simulink model "test_phase_shift_filter"  (R2025b)
settings: Solver=ode1  StartTime=0.0  StopTime=1  FixedStep=ts_inv  RelTol=1e-3
values from neighbouring files (symbols this model uses):
  frequency_set = 300    [init_model_legacy.m]
undefined symbols (not defined in the file or in its folder): ts_inv
libraries: phase_shift_filter x1
settings Model: SimulationMode=accelerator  Creator=dbagn  LastModifiedBy=dbagn
settings SFSimCC: SimCustomHeaderCode=|
  | #include "rpi.h"
  | #include "mavgflt.h"
  | #include "mavgflt_simulink.h"
  | #include "mavgflts.h"
  | #include "mavgflts_simulink.h"
  | #include "dsmavgflt.h"
  | #include "dsmavgflt_simulink.h"
  | #include "bemf_obsv.h"
  | #include "bemf_obsv_simulink.h"
  | #include "bemf_obsv_load_est.h"
  | #include "bemf_obsv_load_est_simulink.h"
  | #include "dqvector_pi.h"
  | #include "dqvector_pi_simulink.h"
  | #include "sv_pwm_simulink.h"
  | #include "sv_pwm.h"
  | #include "first_harmonic_tracker.h"
  | #include "first_harmonic_tracker_simulink.h"
  | #include "dqpll_thyr.h"
  | #include "dqpll_thyr_simulink.h"
  | #include "dqpll_grid.h"
  | #include "dqpll_grid_simulink.h"
  | #include "phase_shift_flt_simulink.h"
  | #include "phase_shift_flt.h"
settings SFSimCC: SimUserSources=|
  | "rpi.c"
  | "mavgflt_simulink.c"
  | "mavgflt.c"
  | "mavgflts_simulink.c"
  | "mavgflts.c"
  | "dsmavgflt_simulink.c"
  | "dsmavgflt.c"
  | "bemf_obsv_simulink.c"
  | "bemf_obsv.c"
  | "bemf_obsv_load_est_simulink.c"
  | "bemf_obsv_load_est.c"
  | "dqvector_pi.c"
  | "dqvector_pi_simulink.c"
  | "sv_pwm_simulink.c"
  | "sv_pwm.c"
  | "first_harmonic_tracker_simulink.c"
  | "first_harmonic_tracker.c"
  | "dqpll_thyr_simulink.c"
  | "dqpll_thyr.c"
  | "dqpll_grid_simulink.c"
  | "dqpll_grid.c"
  | "phase_shift_flt_simulink.c"
  | "phase_shift_flt.c"
settings SFSimCC: SimUserIncludeDirs=|
  | include
  | src

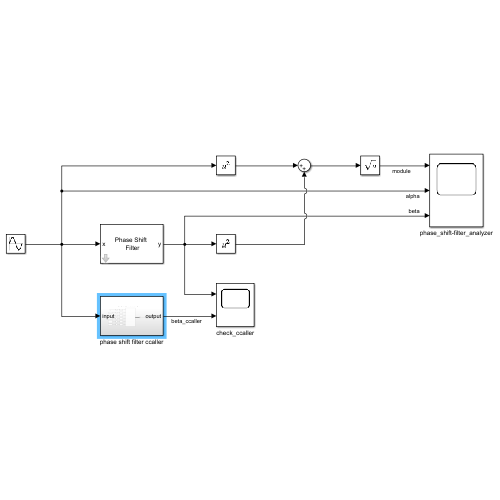
[thumbnail: Simulink's stored preview of the top-level diagram]
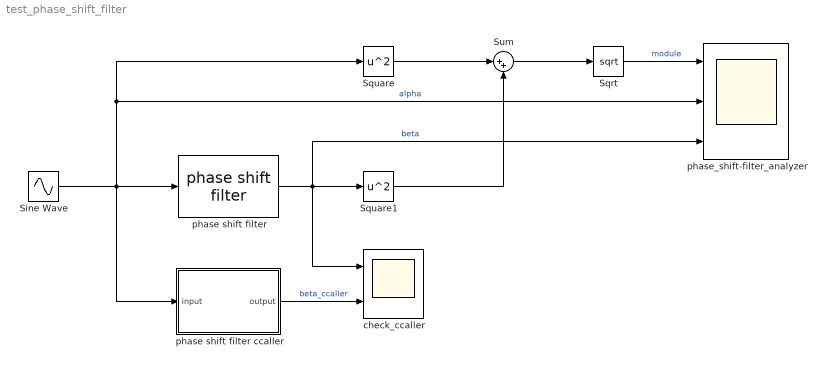
== system test_phase_shift_filter ==
  Sine Wave : Sin  Frequency=frequency_set*2*pi  SampleTime=0
  Sqrt : Sqrt
  Square : Math  Operator=square
  Square1 : Math  Operator=square
  Sum : Sum  Inputs=|++
  check_ccaller : Scope  NumInputPorts=2
      settings: SampleTime=ts_inv  ActiveDisplayYMinimum=-1.2559883330074681  ActiveDisplayYMaximum=1.2979435207382621
  phase shift filter : phase_shift_filter/phase shift filter  f=frequency_set  scaling_factor=phase_shift_filter_gain  ts=ts_inv
  phase shift filter ccaller : Subsystem
  phase_shift-filter_analyzer : Scope  NumInputPorts=3
      settings: SampleTime=ts_inv  ActiveDisplayYMinimum=-1.1297586136004538  ActiveDisplayYMaximum=1.507573484556453
  wires:
  Sine Wave/1 -> phase shift filter ccaller/1(input), Square/1, phase_shift-filter_analyzer/2, phase shift filter/1  "alpha"
  phase shift filter/1 -> check_ccaller/1, phase_shift-filter_analyzer/3, Square1/1  "beta"
  Square/1 -> Sum/1
  Square1/1 -> Sum/2
  Sum/1 -> Sqrt/1
  Sqrt/1 -> phase_shift-filter_analyzer/1  "module"
  phase shift filter ccaller/1(output) -> check_ccaller/2  "beta_ccaller"

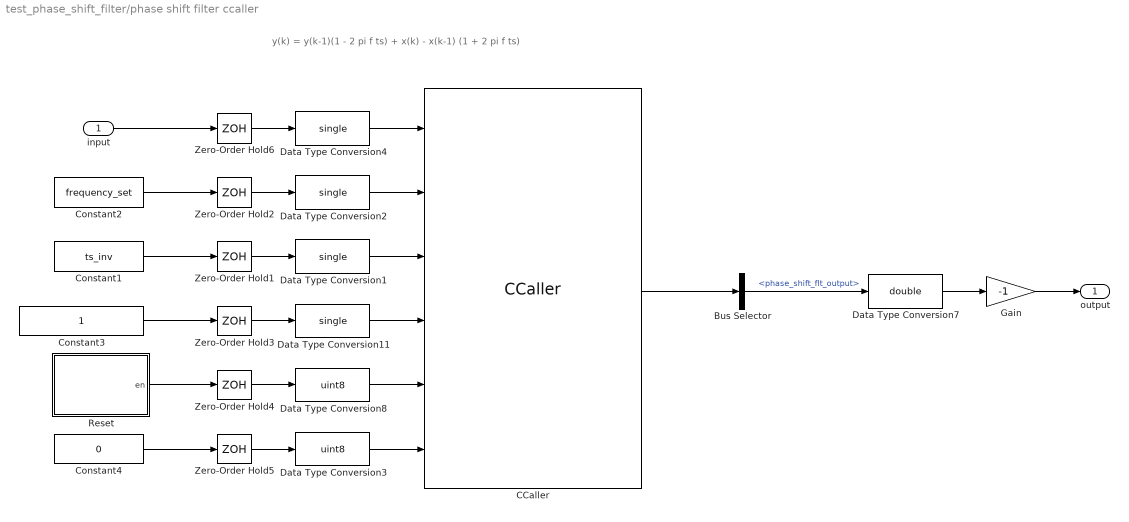
== system test_phase_shift_filter/phase shift filter ccaller ==
  note: y(k) = y(k-1)(1 - 2 pi f ts) + x(k) - x(k-1) (1 + 2 pi f ts)
  input : Inport
  Bus Selector : BusSelector  OutputSignals=phase_shift_flt_output
  CCaller : CCaller  FunctionName=phase_shift_flt_process_simulink  PortSpecificationStruct="%)30     .    , P   8    (     @         %    \"     <    !     0         %  0 \"0    $    _    07)G3F%M90  4&]R=$YA;64 4V-O<&4     26YD97@     5'EP90      4VEZ90      27-';&]B86P   X    P    !@    @    $          4    (     0    ,    !         !   P!O=70 #@   #     &    \"     0         !0    @    !     P    $         $  # &]U=  .    .     8    (    !          %    \"     $    &     0         0   ...(+3823 chars)"  SampleTime=ts_inv
  Constant1 : Constant  Value=ts_inv
  Constant2 : Constant  Value=frequency_set
  Constant3 : Constant
  Constant4 : Constant  Value=0
  Data Type Conversion{1..2,4,11} (4 alike) : DataTypeConversion  OutDataTypeStr=single  SaturateOnIntegerOverflow=off  RndMeth=Floor
  Data Type Conversion3 : DataTypeConversion  OutDataTypeStr=uint8  SaturateOnIntegerOverflow=off  RndMeth=Floor
  Data Type Conversion7 : DataTypeConversion  OutDataTypeStr=double  SaturateOnIntegerOverflow=off  RndMeth=Floor
  Data Type Conversion8 : DataTypeConversion  OutDataTypeStr=uint8  SaturateOnIntegerOverflow=off  RndMeth=Floor
  Gain : Gain  Gain=-1
  Reset : Subsystem
  Zero-Order Hold{1..6} (6 alike) : ZeroOrderHold  SampleTime=ts_inv
  output : Outport
  wires:
  input/1 -> Zero-Order Hold6/1
  Data Type Conversion11/1 -> CCaller/4
  Zero-Order Hold3/1 -> Data Type Conversion11/1
  Constant3/1 -> Zero-Order Hold3/1
  Zero-Order Hold4/1 -> Data Type Conversion8/1
  Reset/1(en) -> Zero-Order Hold4/1
  Data Type Conversion7/1 -> Gain/1
  Data Type Conversion8/1 -> CCaller/5
  Constant1/1 -> Zero-Order Hold1/1
  Zero-Order Hold1/1 -> Data Type Conversion1/1
  Data Type Conversion1/1 -> CCaller/3
  Zero-Order Hold2/1 -> Data Type Conversion2/1
  Constant2/1 -> Zero-Order Hold2/1
  Data Type Conversion2/1 -> CCaller/2
  Zero-Order Hold5/1 -> Data Type Conversion3/1
  Data Type Conversion3/1 -> CCaller/6
  Constant4/1 -> Zero-Order Hold5/1
  CCaller/1 -> Bus Selector/1
  Bus Selector/1 -> Data Type Conversion7/1  "<phase_shift_flt_output>"
  Data Type Conversion4/1 -> CCaller/1
  Gain/1 -> output/1
  Zero-Order Hold6/1 -> Data Type Conversion4/1

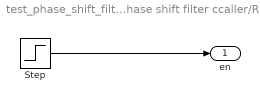
== system test_phase_shift_filter/phase shift filter ccaller/Reset ==
  Step : Step  Time=0.05  Before=1  After=0  SampleTime=ts_inv
  en : Outport
  wires:
  Step/1 -> en/1
